simulink model "aircraft_model"  (R2017a)
settings: Solver=ode4  StartTime=0.0  StopTime=tf  FixedStep=dt  RelTol=1e-3
undefined symbols (not defined in the file): bet_c, d2r, dt, g, gamma_c, omega_n, ph_c, sigbuilder_block, SPEC, u_trim, VT_c, zeta
libraries: sharedtransform x2
settings Model: Creator=FDCL  LastModifiedBy=Jihoon Lee
settings DataIOCC: LimitDataPoints=on  SaveFormat=Array  SignalLoggingSaveFormat=ModelDataLogs
settings OptimizationCC: BlockReduction=off  BooleanDataType=off  LifeSpan=inf
settings DebuggingCC: SaveWithParameterizedLinksMsg=none  UnderspecifiedInitializationDetection=Classic  MergeDetectMultiDrivingBlocksExec=none  MultiTaskDSMMsg=warning  MultiTaskCondExecSysMsg=none  StateNameClashWarn=warning  SFUnexpectedBacktrackingDiag=warning  SFNoUnconditionalDefaultTransitionDiag=warning  SFExecutionAtInitializationDiag=none
settings HardwareCC: ProdBitPerPointer=32  ProdBitPerSizeT=32  ProdBitPerPtrDiffT=32  ProdLargestAtomicFloat=None  ProdIntDivRoundTo=Undefined  ProdEndianess=Unspecified  ProdWordSize=32  ProdHWDeviceType=32-bit Generic  TargetBitPerPointer=64  TargetBitPerSizeT=64  TargetBitPerPtrDiffT=64  TargetLongLongMode=on  TargetIntDivRoundTo=Zero  TargetEndianess=LittleEndian  TargetWordSize=64  TargetHWDeviceType=MATLAB Host  ProdEqTarget=off
settings ModelReferenceCC: PropagateSignalLabelsOutOfModel=off
settings GRTTargetCC: TargetLangStandard=C89/C90 (ANSI)  GeneratePreprocessorConditionals=Disable all
settings ConfigComp: CovMetricSettings=dw  CovHtmlReporting=on  CovSaveCumulativeToWorkspaceVar=on  CovSaveSingleToWorkspaceVar=on  CovExternalEMLEnable=off

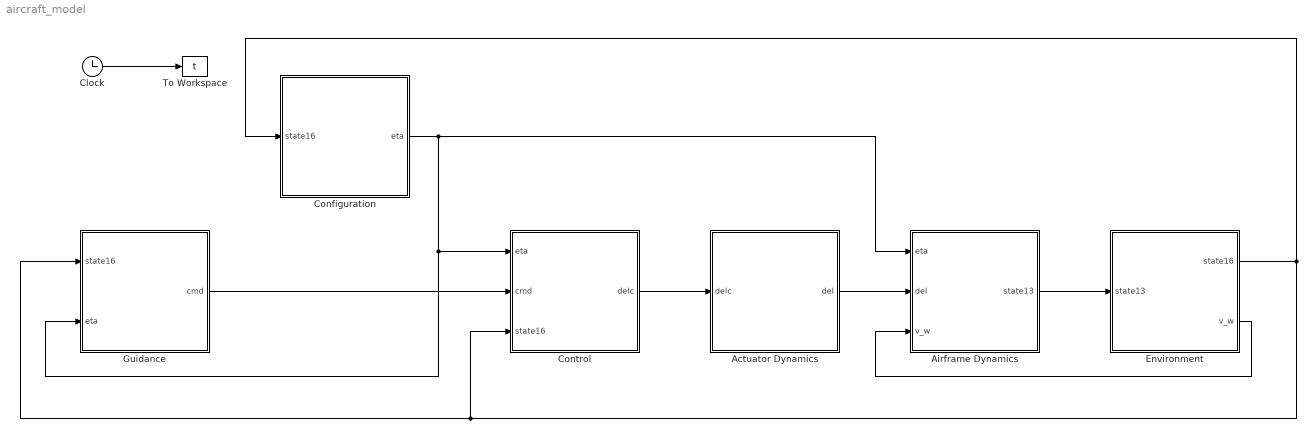
== system aircraft_model ==
  Actuator Dynamics : Subsystem  TreatAsAtomicUnit=on
  Airframe Dynamics : Subsystem
  Clock : Clock
  Configuration : Subsystem  VariantControl=scnMorph==1
  Control : Subsystem  TreatAsAtomicUnit=on  VariantControl=ndiExact==1
  Environment : Subsystem
  Guidance : Subsystem  VariantControl=scnMorph==1
  To Workspace : ToWorkspace  VariableName=t  SampleTime=-1
  wires:
  Clock/1 -> To Workspace/1
  Configuration/1(eta) -> Airframe Dynamics/1(eta), Control/1(eta), Guidance/2(eta)
  Control/1(delc) -> Actuator Dynamics/1(delc)
  Actuator Dynamics/1(del) -> Airframe Dynamics/2(del)
  Guidance/1(cmd) -> Control/2(cmd)
  Airframe Dynamics/1(state13) -> Environment/1(state13)
  Environment/2(v_w) -> Airframe Dynamics/3(v_w)
  Environment/1(state16) -> Control/3(state16), Guidance/1(state16), Configuration/1(state16)

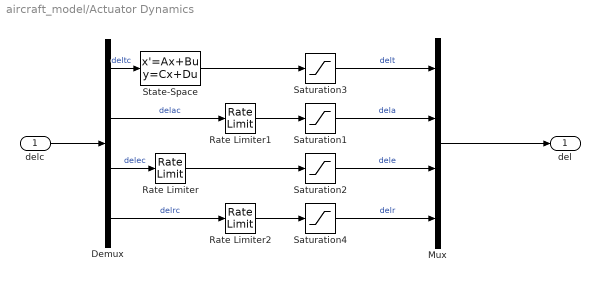
== system aircraft_model/Actuator Dynamics ==
  delc : Inport  OutDataTypeStr=double  PortDimensions=[4 1]  SampleTime=dt
  Demux : Demux
  Mux : Mux
  Rate Limiter : RateLimiter  RisingSlewLimit=40*d2r  FallingSlewLimit=-40*d2r  SampleTimeMode=inherited  InitialCondition=u_trim(3)
  Rate Limiter1 : RateLimiter  RisingSlewLimit=100*d2r  FallingSlewLimit=-100*d2r  SampleTimeMode=inherited  InitialCondition=u_trim(2)
  Rate Limiter2 : RateLimiter  RisingSlewLimit=82*d2r  FallingSlewLimit=-82*d2r  SampleTimeMode=inherited  InitialCondition=u_trim(4)
  Saturation1 : Saturate  UpperLimit=SPEC.dela_ul  LowerLimit=SPEC.dela_ll
  Saturation2 : Saturate  UpperLimit=SPEC.dele_ul  LowerLimit=SPEC.dele_ll
  Saturation3 : Saturate  UpperLimit=1  LowerLimit=0
  Saturation4 : Saturate  UpperLimit=SPEC.delr_ul  LowerLimit=SPEC.delr_ll
  State-Space : StateSpace  A=[0 1; -omega_n^2 -2*zeta*omega_n]  B=[0; omega_n^2]  C=[1 0]  D=0  X0=u_trim(1)
  del : Outport  OutDataTypeStr=double  PortDimensions=[4 1]  SampleTime=dt
  wires:
  Rate Limiter1/1 -> Saturation1/1
  Demux/2 -> Rate Limiter1/1  "delac"
  Rate Limiter2/1 -> Saturation4/1
  Demux/3 -> Rate Limiter/1  "delec"
  Demux/1 -> State-Space/1  "deltc"
  Demux/4 -> Rate Limiter2/1  "delrc"
  Saturation3/1 -> Mux/1  "delt"
  Saturation2/1 -> Mux/3  "dele"
  Saturation1/1 -> Mux/2  "dela"
  Saturation4/1 -> Mux/4  "delr"
  delc/1 -> Demux/1
  Mux/1 -> del/1
  State-Space/1 -> Saturation3/1
  Rate Limiter/1 -> Saturation2/1

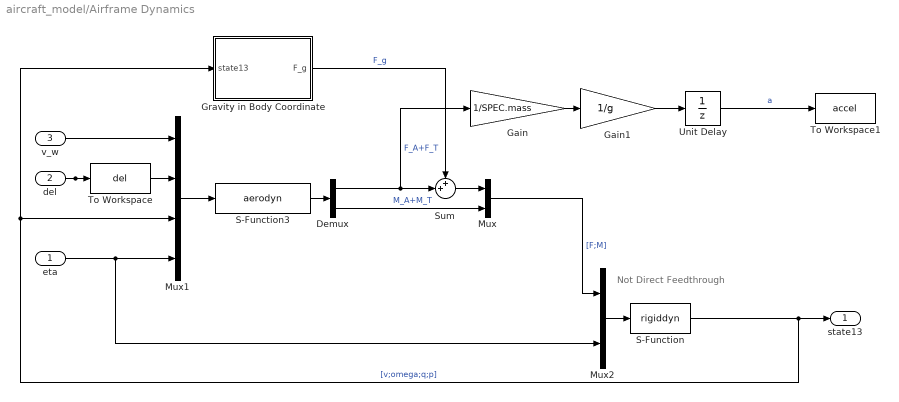
== system aircraft_model/Airframe Dynamics ==
  note: Not Direct
      | Feedthrough
  eta : Inport  PortDimensions=[2 1]  SampleTime=dt
  del : Inport  Port=2  PortDimensions=[4 1]  SampleTime=dt
  v_w : Inport  Port=3  Unit=m/s  PortDimensions=[3 1]  SampleTime=dt
  Demux : Demux  Outputs=[3 3]
  Gain : Gain  Gain=1/SPEC.mass
  Gain1 : Gain  Gain=1/g
  Gravity in Body Coordinate : Subsystem  TreatAsAtomicUnit=on
  Mux : Mux  Inputs=[3 3]
  Mux1 : Mux  Inputs=[3 4 13 2]
  Mux2 : Mux  Inputs=[6 2]
  S-Function : S-Function  FunctionName=rigiddyn  Parameters=state130  SFunctionDeploymentMode=off  EnableBusSupport=off
  S-Function3 : S-Function  FunctionName=aerodyn  SFunctionDeploymentMode=off  EnableBusSupport=off
  Sum : Sum  Inputs=++|
  To Workspace : ToWorkspace  VariableName=del  SampleTime=-1
  To Workspace1 : ToWorkspace  VariableName=accel  SampleTime=-1
  Unit Delay : UnitDelay  InitialCondition=[0;0;0]  SampleTime=dt
  state13 : Outport  PortDimensions=[13 1]  SampleTime=dt
  wires:
  S-Function3/1 -> Demux/1
  Gain1/1 -> Unit Delay/1
  Gain/1 -> Gain1/1
  Demux/2 -> Mux/2  "M_A+M_T"
  Sum/1 -> Mux/1
  Demux/1 -> Sum/2, Gain/1  "F_A+F_T"
  Mux/1 -> Mux2/1  "[F;M]"
  eta/1 -> Mux2/2, Mux1/4
  Mux2/1 -> S-Function/1
  Mux1/1 -> S-Function3/1
  v_w/1 -> Mux1/1
  S-Function/1 -> state13/1, Mux1/3, Gravity in Body Coordinate/1(state13)  "[v;omega;q;p]"
  Gravity in Body Coordinate/1(F_g) -> Sum/1  "F_g"
  Unit Delay/1 -> To Workspace1/1  "a"
  del/1 -> Mux1/2, To Workspace/1

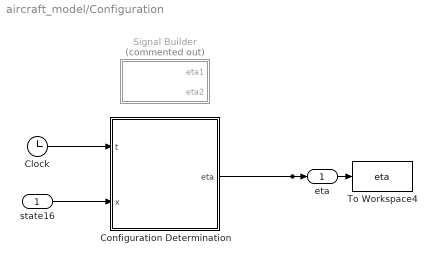
== system aircraft_model/Configuration ==
  state16 : Inport  PortDimensions=[16 1]  SampleTime=dt
  Clock : Clock
  Configuration Determination : MATLAB Function  TreatAsAtomicUnit=on
  Signal Builder : Subsystem  Tag=STV Subsys  Commented=on  LoadFcn=sigbuilder_block('load');  StartFcn=sigbuilder_block('start');  StopFcn=sigbuilder_block('stop');  ClipboardFcn=sigbuilder_block('clipboard');  mask(Sigbuilder block){tuvar=[0:10]}
      mask help: Simulink:masks:SigbuilderBlock_MD
      mask init:
      | if ~strcmp(get_param(bdroot(gcbh),'SimulationStatus'),'stopped') tuvar = sigbuilder_block('maskInit'); end
      settings: CopyFcn=sigbuilder_block('copy');  DeleteFcn=sigbuilder_block('delete');  ModelCloseFcn=sigbuilder_block('modelClose');  PreSaveFcn=sigbuilder_block('preSave');  PauseFcn=sigbuilder_block('pause');  ContinueFcn=sigbuilder_block('continue');  NameChangeFcn=sigbuilder_block('namechange');  OpenFcn=sigbuilder_block('open',[176.25 153.75 550.5 358.5 ]);  CloseFcn=sigbuilder_block('close');
      mask Display: plot(0, 0, 100, 100,[2, 2, 32, 32, 2], [68, 8, 8, 68, 68],[32, 2], [38, 38], [32, 19, 2],[53, 60, 44], [32, 17, 17, 2],[16, 16, 31, 31]);txt = getActiveGroup(gcbh);text(2, 100, txt,'verticalAlignment', 'top');
  To Workspace4 : ToWorkspace  VariableName=eta  SampleTime=-1
  eta : Outport  PortDimensions=[2 1]  SampleTime=dt
  wires:
  Configuration Determination/1(eta) -> To Workspace4/1, eta/1
  state16/1 -> Configuration Determination/2(x)
  Clock/1 -> Configuration Determination/1(t)

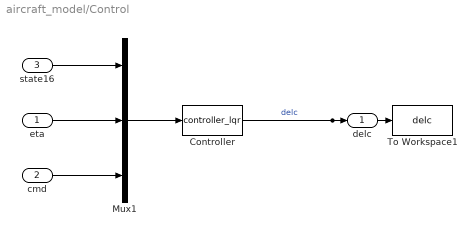
== system aircraft_model/Control ==
  eta : Inport  PortDimensions=[2 1]  SampleTime=dt
  cmd : Inport  Port=2  PortDimensions=[4 1]  SampleTime=dt
  state16 : Inport  Port=3  PortDimensions=[16 1]  SampleTime=dt
  Controller : S-Function  FunctionName=controller_lqr  Parameters=param  SFunctionDeploymentMode=off  EnableBusSupport=off
  Mux1 : Mux  Inputs=[16 2 4]
  To Workspace1 : ToWorkspace  VariableName=delc  SampleTime=-1
  delc : Outport  PortDimensions=[4 1]  SampleTime=dt
  wires:
  Controller/1 -> To Workspace1/1, delc/1  "delc"
  state16/1 -> Mux1/1
  eta/1 -> Mux1/2
  cmd/1 -> Mux1/3
  Mux1/1 -> Controller/1

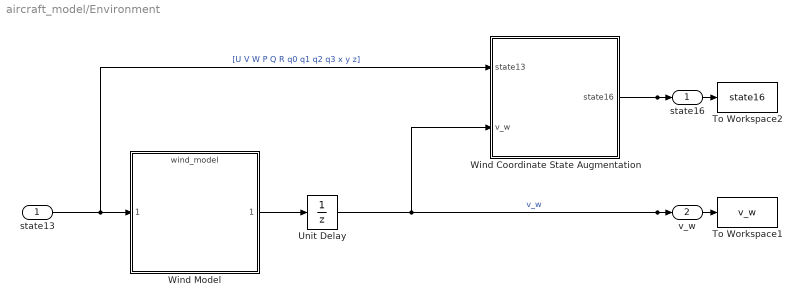
== system aircraft_model/Environment ==
  state13 : Inport
  To Workspace1 : ToWorkspace  VariableName=v_w  SampleTime=-1
  To Workspace2 : ToWorkspace  VariableName=state16  SampleTime=-1
  Unit Delay : UnitDelay  InitialCondition=[0;0;0]  SampleTime=-1
  Wind Coordinate State Augmentation : Subsystem
  Wind Model : ModelReference  ModelNameDialog=wind_model  SimulationMode=Normal  ModelReferenceVersion=1.78
  state16 : Outport  PortDimensions=[16 1]  SampleTime=dt
  v_w : Outport  Port=2  Unit=m/s  PortDimensions=[3 1]  SampleTime=dt
  wires:
  Unit Delay/1 -> Wind Coordinate State Augmentation/2(v_w), To Workspace1/1, v_w/1  "v_w"
  Wind Model/1 -> Unit Delay/1
  state13/1 -> Wind Coordinate State Augmentation/1(state13), Wind Model/1  "[U V W P Q R q0 q1 q2 q3 x y z]"
  Wind Coordinate State Augmentation/1(state16) -> To Workspace2/1, state16/1

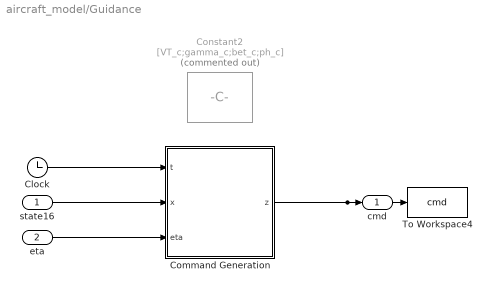
== system aircraft_model/Guidance ==
  state16 : Inport  PortDimensions=[16 1]  SampleTime=dt
  eta : Inport  Port=2  PortDimensions=[2 1]  SampleTime=dt
  Clock : Clock
  Command Generation : MATLAB Function  TreatAsAtomicUnit=on
  Constant2 : Constant  Commented=on  Value=[VT_c;gamma_c;bet_c;ph_c]  VectorParams1D=off
  To Workspace4 : ToWorkspace  VariableName=cmd  SampleTime=-1
  cmd : Outport  PortDimensions=[4 1]  SampleTime=dt
  wires:
  Command Generation/1(z) -> cmd/1, To Workspace4/1
  state16/1 -> Command Generation/2(x)
  eta/1 -> Command Generation/3(eta)
  Clock/1 -> Command Generation/1(t)

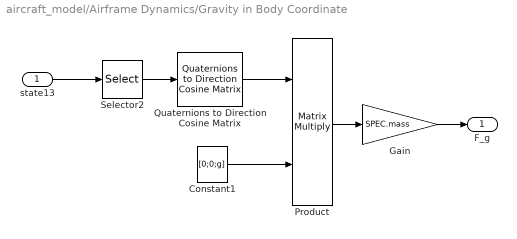
== system aircraft_model/Airframe Dynamics/Gravity in Body Coordinate ==
  state13 : Inport  PortDimensions=[13 1]  SampleTime=dt
  Constant1 : Constant  Value=[0;0;g]  VectorParams1D=off  SampleTime=dt
  Gain : Gain  Gain=SPEC.mass
  Product : Product  Multiplication=Matrix(*)
  Quaternions to Direction Cosine Matrix : sharedtransform/Quaternions to  Direction Cosine Matrix
      settings: SourceProductName=Aerospace Blockset  SourceProductBaseCode=AE
  Selector2 : Selector  InputPortWidth=13  IndexOptions=Index vector (dialog)  Indices=7:10  OutputSizes=1
  F_g : Outport  Unit=N  PortDimensions=[3 1]  SampleTime=dt
  wires:
  state13/1 -> Selector2/1
  Gain/1 -> F_g/1
  Product/1 -> Gain/1
  Selector2/1 -> Quaternions to Direction Cosine Matrix/1
  Quaternions to Direction Cosine Matrix/1 -> Product/1
  Constant1/1 -> Product/2

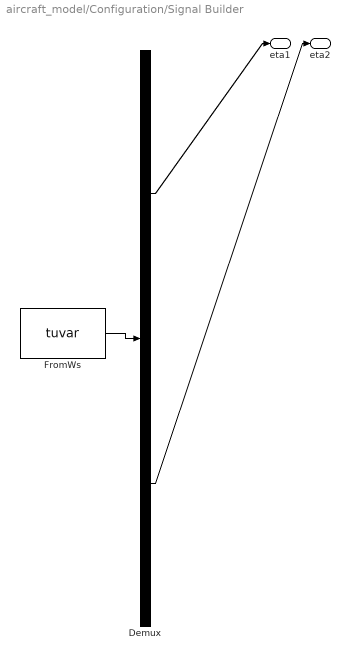
== system aircraft_model/Configuration/Signal Builder ==
  Demux : Demux  Tag=STV Demux  Outputs=2
  FromWs : FromWorkspace  Tag=STV FromWs  VariableName=tuvar  SampleTime=0
      SigBuilderData=|
      | common.afterFinalStr = 'Extrapolate'
      | common.sampleTime = 0
      | dataSet(1).timeRange = [0 100]
      | dataSet(1).name = 'Group 1'
      | dataSet(2).timeRange = [0 30]
      | dataSet(2).name = 'Group 2'
      | sbobj.Groups(1).Name = 'Group 1'
      | sbobj.Groups(1).Signals(1).Name = 'eta1'
      | sbobj.Groups(1).Signals(1).XData = [0 10 11 20 21 30 31 40 41 50 51 100]
      | sbobj.Groups(1).Signals(1).YData = [0 0 0.25 0.25 0.5 0.5 0.75 0.75 1 1 0.5 0.5]
      | sbobj.Groups(1).Signals(2).Name = 'eta2'
      | sbobj.Groups(1).Signals(2).XData = [0 1 1 2 2 3 3 4 4 5 5 6 6 7 7 8 8 9 9 10 10 11 11 12 12 13 13 14 14 15 15 16 16 17 17 18 18 19 19 20 20 21 21 22 22 23 23 24 24 25 25 26 26 27 27 28 28 29 29 30 30 31 31 32 32 33 33 34 34 35 35 36 36 37 37 38 38 39 39 40 40 41 41 42 42 43 43 44 44 45 45 46 46 47 47 48 48 49 49 50 50 51 51 52 52 53 53 54 54 55 55 56 56 57 57 58 58 59 59 60 60 61 61 62 62 63 63 64 64 65 65 66 66 67 67 68 68 69 69 70 70 71 71 72 72 73 73 74 74 75 75 76 76 77 77 78 78 79 79 80 80 81 81 82 82 83 83 84 84 85 85 86 86 87 87 88 88 89 89 90 90 91 91 92 92 93 93 94 94 95 95 96 96 97 97 98 98 99 99 100 100]
      | sbobj.Groups(1).Signals(2).YData = [0 2 0 2 0 2 0 2 0 2 0 2 0 2 0 2 0 2 0 2 0 2 0 2 0 2 0 2 0 2 0 2 0 2 0 2 0 2 0 2 0 2 0 2 0 2 0 2 0 2 0 2 0 2 0 2 0 2 0 2 0 2 0 2 0 2 0 2 0 2 0 2 0 2 0 2 0 2 0 2 0 2 0 2 0 2 0 2 0 2 0 2 0 2 0 2 0 2 0 2 0 2 0 2 0 2 0 2 0 2 0 2 0 2 0 2 0 2 0 2 0 2 0 2 0 2 0 2 0 2 0 2 0 2 0 2 0 2 0 2 0 2 0 2 0 2 0 2 0 2 0 2 0 2 0 2 0 2 0 2 0 2 0 2 0 2 0 2 0 2 0 2 0 2 0 2 0 2 0 2 0 2 0 2 0 2 0 2 0 2 0 2 0 2 0 2 0 2 0 2 0]
      | sbobj.Groups(1).TimeRange = [0 100]
      | sbobj.Groups(2).Name = 'Group 2'
      | sbobj.Groups(2).Signals(1).Name = 'eta1'
      | sbobj.Groups(2).Signals(1).XData = [0 20 20 30]
      | sbobj.Groups(2).Signals(1).YData = [0 0 1 1]
      | sbobj.Groups(2).Signals(2).Name = 'eta2'
      | sbobj.Groups(2).Signals(2).XData = [0 10 10 30]
      | sbobj.Groups(2).Signals(2).YData = [0 0 1 1]
      | sbobj.Groups(2).TimeRange = [0 30]
  eta1 : Outport  Tag=STV Outport
  eta2 : Outport  Tag=STV Outport  Port=2
  wires:
  FromWs/1 -> Demux/1
  Demux/1 -> eta1/1
  Demux/2 -> eta2/1

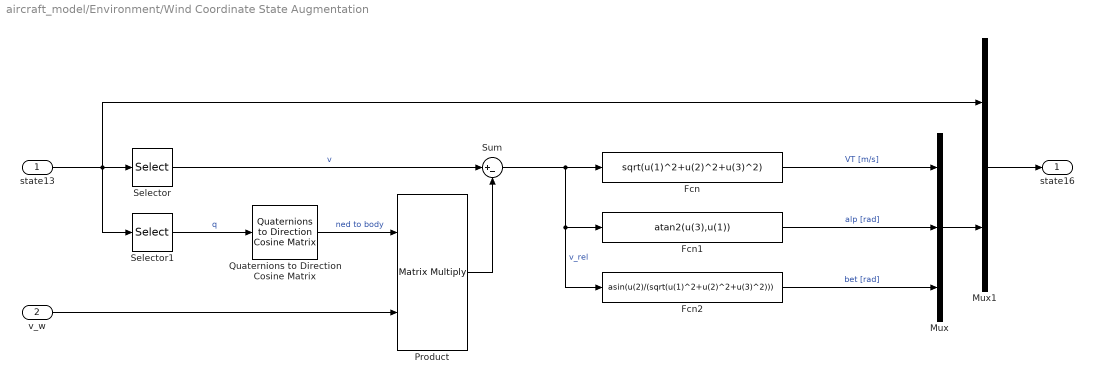
== system aircraft_model/Environment/Wind Coordinate State Augmentation ==
  state13 : Inport  OutDataTypeStr=double  PortDimensions=[13 1]  SampleTime=dt
  v_w : Inport  Port=2  OutDataTypeStr=double  Unit=m/s  PortDimensions=[3 1]  SampleTime=dt
  Fcn : Fcn  Expr=sqrt(u(1)^2+u(2)^2+u(3)^2)
  Fcn1 : Fcn  Expr=atan2(u(3),u(1))
  Fcn2 : Fcn  Expr=asin(u(2)/(sqrt(u(1)^2+u(2)^2+u(3)^2)))
  Mux : Mux  Inputs=3
  Mux1 : Mux  Inputs=[13 3]
  Product : Product  Multiplication=Matrix(*)
  Quaternions to Direction Cosine Matrix : sharedtransform/Quaternions to  Direction Cosine Matrix
      settings: SourceProductName=Aerospace Blockset  SourceProductBaseCode=AE
  Selector : Selector  InputPortWidth=13  IndexOptions=Index vector (dialog)  Indices=[1:3]  OutputSizes=1
  Selector1 : Selector  InputPortWidth=13  IndexOptions=Index vector (dialog)  Indices=[7:10]  OutputSizes=1
  Sum : Sum  Inputs=|+-
  state16 : Outport  OutDataTypeStr=double  PortDimensions=[16 1]  SampleTime=dt
  wires:
  Quaternions to Direction Cosine Matrix/1 -> Product/1  "ned to body"
  Sum/1 -> Fcn/1, Fcn1/1, Fcn2/1  "v_rel"
  v_w/1 -> Product/2
  Selector/1 -> Sum/1  "v"
  state13/1 -> Selector/1, Selector1/1, Mux1/1
  Fcn1/1 -> Mux/2  "alp [rad]"
  Product/1 -> Sum/2
  Selector1/1 -> Quaternions to Direction Cosine Matrix/1  "q"
  Fcn/1 -> Mux/1  "VT [m/s]"
  Fcn2/1 -> Mux/3  "bet [rad]"
  Mux1/1 -> state16/1
  Mux/1 -> Mux1/2

== matlab function aircraft_model/Configuration/Configuration Determination ==
  data: t input; x input; eta output
function eta = config(t,x)

T = 0:10:50;
Eta = [0 1 1 0 0; % span
       0 0 1 1 0]; % sweep

eta = zeros(2,1);

if (t >= T(1))&&(t < T(2))
    eta = Eta(:,1);
elseif (t >= T(2))&&(t < T(3))
    eta = Eta(:,2);
elseif (t >= T(3))&&(t < T(4))
    eta = Eta(:,3);
elseif (t >= T(4))&&(t < T(5))
    eta = Eta(:,4);
elseif t >= T(5)
    eta = Eta(:,5);
end

== matlab function aircraft_model/Guidance/Command Generation ==
  data: t input; x input; z output; eta input
function z = gen_command(t,x,eta)

z = zeros(4,1);

T = 0:10:50;
Z = zeros(2,length(T)-1);
Z(1,:) = [20 18 20 25 20]; % airspeed command [m/s]
Z(2,:) = [0  3  0 -3  0]*pi/180; % fpa command [rad]

if (t >= T(1))&&(t < T(2))
    z(1:2) = Z(:,1);
elseif (t >= T(2))&&(t < T(3))
    z(1:2) = Z(:,2);
elseif (t >= T(3))&&(t < T(4))
    z(1:2) = Z(:,3);
elseif (t >= T(4))&&(t < T(5))
    z(1:2) = Z(:,4);
elseif t >= T(5)
    z(1:2) = Z(:,5);
end
